simulink model "gmp_pmsm_sensored_nonlinear_sil_mdl_2022b"  (R2022b)
settings: Solver=VariableStepAuto  StartTime=0.0  StopTime=10  RelTol=1e-3
model workspace (MAT data in the model file):
  B = 0
  BW_i = 800
  Flux_t = 0.12
  IQ24 : Simulink.NumericType (value not decoded)
  J = 0.018
  K_d = 3.72061852168
  K_m = 0.128242020589
  K_u = 0.00236407598332
  Ki_id = 0.001
  Ki_iq = 1
  Ki_n = 25225.1136556
  Kp_id = 1e-05
  Kp_iq = 5e-05
  Kp_n = 12.6125568278
  Ld_t = 0.00303
  Lq_t = 0.02019
  Max_p = 0.006000830667
  P = 2
  RLS_ini_a = 1000000
  Rd_mos = 0.01
  Rs = 0.1215
  Rv = 6.4
  T_final = 0
  T_initial = 0
  Tes = [4 7 10 7 4]
  Tf_t = 0.1
  Tm = 0
  Udq_limit = 550
  Var = 0
  Vce0 = 0
  Vd0 = 0
  Vdc = 80
  button = 1
  im_limit = 40
  mean_prd = 10
  position_init = 0.2
  r_ce = 1e-08
  r_d = 1e-08
  sample_prd = 100
  step_time = 0.2
  ts = 6.25e-05
  wc = 3500
libraries: peripheral_utilities x9, spsSeriesRLCBranchLib x6, spsMosfetLib x6, simulink x3, spsVoltageMeasurementLib x2, gmp_sil_core_pack x1, spsPermanentMagnetSynchronousMachineLib x1, spsdq0toabcLib x1, spsFourierLib x1, spsControlledVoltageSourceLib x1, sps_lib x1
(part 2 of 3)

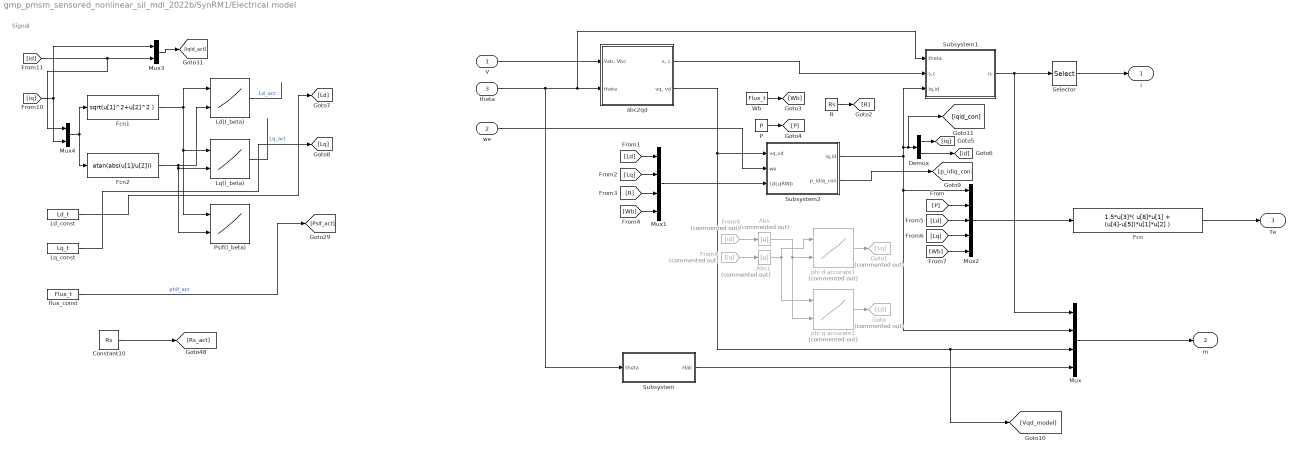
== system gmp_pmsm_sensored_nonlinear_sil_mdl_2022b/SynRM1/Electrical model ==
  note: Signal
  V : Inport
  we : Inport  Port=2
  theta : Inport  Port=3
  Abs : Abs  Commented=on  SaturateOnIntegerOverflow=off
  Abs1 : Abs  Commented=on  SaturateOnIntegerOverflow=off
  Constant10 : Constant  Value=Rs
  Demux : Demux  Outputs=2
  Fcn : Fcn  Expr=1.5*u[3]*( u[6]*u[1] + (u[4]-u[5])*u[1]*u[2] )
  Fcn1 : Fcn  Expr=sqrt(u[1]^2+u[2]^2 )
  Fcn2 : Fcn  Expr=atan(abs(u[1]/u[2]))
  From8 : From  Commented=on  GotoTag=iq
  From9 : From  Commented=on  GotoTag=id
  Goto : Goto  Commented=on  GotoTag=Ld
  Goto1 : Goto  Commented=on  GotoTag=Lq
  Ld(I_beta) : Lookup_n-D  BreakpointsForDimension1=[0,4,8,12,16,20,24,28,32,36,40,44,48,52,56,60,64,68,72,76]  BreakpointsForDimension2=[0,4,8,12,16,20,24,28,32,36,40,44,48,52,56,60,64,68,72,76,80,84,88,90]  Table=[0.0090049,0.0090049,0.0090049,0.0090049,0.0090049,0.0090049,0.0090049,0.0090049,0.0090049,0.0090049,0.0090049,0.0090049,0.0090049,0.0090049,0.0090049,0.0090049,0.0090049,0.0090049,0.0090049,0.0090049,0.0090049,0.0090049,0.0090049,0.0090049;0.0091068,0.0083359,0.0077182,0.0071952,0.0067602,0.0063986,0.0061075,0.0058615,0.0056442,0.0054621,0.0053073,0.0051722,0.0050586,0.0049576,0.0048709,0.0047948,0.0047272,0.0046738,0.0046308,0.0045967,0.00457,0.0045527,0.0045425,0.0045403;0.0093464,0.0079938,0.0070425,0.006355,0.0058504,0.0054685,0.005168,0.004922,0.0047173,0.0045442,0.0044053,0.0042808,0.0041752,0.0040816,0.0040014,0.0039315,0.0038713,0.0038189,0.0037747,0.0037414,0.0037159,0.0036999,0.0036913,0.0036904;0.0094184,0.0086648,0.007532,0.0065799,0.0059032,0.0053778,0.0049522,0.0046235,0.0043749,0.0041848,0.0040338,0.0039102,0.0038062,0.0037163,0.0036343,0.0035659,0.003505,0.0034522,0.0034077,0.003372,0.0033446,0.0033271,0.0033182,0.003317;0.007537,0.0073523,0.0068251,0.0060935,0.0054955,0.0050421,0.0046797,0.0043924,0.0041627,0.0039813,0.0038382,0.003715,0.0036051,0.0035122,0.0034334,0.0033641,0.0033014,0.0032455,0.0031985,0.00316,0.0031309,0.0031118,0.0031022,0.0031011;0.0069136,0.0066119,0.0061429,0.0055601,0.0050595,0.0046689,0.004363,0.0041106,0.0039094,0.0037548,0.0036311,0.0035297,0.003445,0.0033686,0.0032942,0.0032267,0.0031671,0.0031114,0.0030613,0.0030204,0.0029894,0.002969,0.0029587,0.0029574;0.0067888,0.0062678,0.005688,0.0051372,0.0047121,0.0043706,0.0040971,0.0038745,0.0037001,0.0035638,0.0034559,0.0033682,0.0032948,0.0032327,0.0031761,0.0031194,0.0030631,0.0030118,0.0029628,0.0029201,0.0028873,0.0028657,0.002855,0.0028536;0.0064852,0.0059179,0.0053416,0.0048215,0.0044208,0.0041168,0.0038718,0.0036757,0.0035267,0.0034084,0.0033126,0.0032335,0.0031693,0.0031162,0.0030692,0.0030242,0.0029766,0.0029286,0.0028841,0.0028423,0.0028087,0.0027864,0.0027753,0.0027739;0.0061523,0.0056113,0.0050565,0.0045719,0.0041984,0.0039199,0.0036926,0.0035158,0.0033808,0.0032752,0.0031919,0.0031227,0.0030647,0.0030165,0.0029765,0.0029393,0.0029008,0.0028583,0.002817,0.002778,0.0027453,0.0027227,0.0027115,0.0027103;0.0058954,0.0053596,0.0048097,0.0043561,0.0040148,0.0037503,0.0035417,0.0033833,0.0032591,0.0031631,0.0030877,0.0030266,0.0029757,0.0029326,0.0028962,0.0028645,0.0028327,0.0027967,0.0027584,0.0027223,0.002691,0.0026694,0.0026587,0.0026572;0.0056976,0.0051489,0.0045961,0.004167,0.0038525,0.0036066,0.0034122,0.0032677,0.0031545,0.0030661,0.0029972,0.0029426,0.0028976,0.0028598,0.0028271,0.0027991,0.0027724,0.0027421,0.002707,0.0026731,0.0026436,0.0026234,0.0026135,0.0026121;0.0055231,0.0049627,0.0044187,0.0040007,0.0037069,0.0034785,0.0032983,0.0031643,0.0030617,0.0029804,0.0029182,0.0028686,0.0028288,0.0027956,0.0027666,0.0027417,0.0027187,0.0026929,0.0026618,0.0026296,0.0026011,0.0025825,0.0025738,0.0025727;0.0053694,0.0047911,0.0042535,0.0038565,0.0035785,0.0033645,0.0031988,0.0030752,0.0029797,0.0029055,0.0028481,0.0028031,0.002767,0.0027377,0.002713,0.0026907,0.0026708,0.0026487,0.0026213,0.0025909,0.0025632,0.0025454,0.0025381,0.0025373;0.0052237,0.0046319,0.0041064,0.0037302,0.0034662,0.0032628,0.0031101,0.0029956,0.0029078,0.0028387,0.0027859,0.0027449,0.0027117,0.0026861,0.0026645,0.0026452,0.0026275,0.0026087,0.0025847,0.002556,0.0025292,0.0025117,0.0025053,0.0025047;0.0050914,0.0044851,0.003973,0.0036151,0.0033625,0.0031734,0.0030322,0.0029247,0.0028431,0.0027797,0.0027305,0.0026924,0.0026625,0.0026388,0.0026201,0.002604,0.0025886,0.0025725,0.0025511,0.0025243,0.0024983,0.0024809,0.0024746,0.0024742;0.004977,0.004351,0.0038492,0.0035074,0.0032708,0.0030953,0.0029629,0.0028607,0.0027852,0.0027265,0.002681,0.0026455,0.0026177,0.0025961,0.0025796,0.0025663,0.0025528,0.0025391,0.0025203,0.0024953,0.00247,0.0024526,0.002446,0.0024453;0.0048627,0.0042246,0.0037365,0.0034117,0.0031881,0.0030249,0.0028998,0.002804,0.0027327,0.0026783,0.0026359,0.0026029,0.0025771,0.0025573,0.0025427,0.0025312,0.0025199,0.0025084,0.0024918 ...(+761 chars)]  InterpMethod=Akima spline  RndMeth=Simplest
      settings: InputPortMap=u0,u1
  Ld_const : Constant  Value=Ld_t
  Lq(I_beta) : Lookup_n-D  BreakpointsForDimension1=[0,4,8,12,16,20,24,28,32,36,40,44,48,52,56,60,64,68,72,76]  BreakpointsForDimension2=[0,4,8,12,16,20,24,28,32,36,40,44,48,52,56,60,64,68,72,76,80,84,88,90]  Table=[0.027272,0.027272,0.027272,0.027272,0.027272,0.027272,0.027272,0.027272,0.027272,0.027272,0.027272,0.027272,0.027272,0.027272,0.027272,0.027272,0.027272,0.027272,0.027272,0.027272,0.027272,0.027272,0.027272,0.027272;0.027457,0.027451,0.027443,0.027434,0.027425,0.027414,0.027402,0.02739,0.027376,0.027361,0.027345,0.027328,0.027312,0.027294,0.027277,0.02726,0.027243,0.027228,0.027214,0.027202,0.027193,0.027187,0.027183,0.027183;0.027424,0.02742,0.027429,0.027443,0.027463,0.027488,0.027502,0.027506,0.027502,0.027489,0.02747,0.027448,0.02742,0.027389,0.027353,0.027315,0.027274,0.027232,0.02719,0.027153,0.027123,0.027102,0.027091,0.02709;0.024416,0.024514,0.024663,0.024863,0.025117,0.025413,0.025742,0.02607,0.026395,0.026688,0.026936,0.027154,0.027312,0.027386,0.02738,0.027348,0.027301,0.027245,0.027182,0.027117,0.027059,0.027015,0.026992,0.026989;0.02017,0.02027,0.02045,0.020689,0.02099,0.021369,0.02182,0.022355,0.022972,0.023672,0.024447,0.025225,0.025912,0.02649,0.026932,0.027211,0.027268,0.027228,0.027161,0.02708,0.026997,0.026928,0.026888,0.026883;0.017083,0.017167,0.017325,0.017546,0.017836,0.018192,0.018626,0.019145,0.019755,0.020476,0.021306,0.02226,0.023328,0.024442,0.025444,0.02627,0.026871,0.027127,0.027109,0.027029,0.026931,0.026839,0.026782,0.026775;0.014717,0.014798,0.014939,0.015143,0.015413,0.015756,0.016171,0.016667,0.017254,0.017938,0.018741,0.019678,0.02076,0.022,0.023359,0.024679,0.025792,0.026628,0.026978,0.026954,0.026855,0.026746,0.026674,0.026664;0.012887,0.012961,0.013093,0.013279,0.013524,0.013837,0.014221,0.014684,0.015243,0.015903,0.016678,0.017574,0.018624,0.019853,0.021269,0.022834,0.024363,0.025653,0.026571,0.02683,0.026764,0.026648,0.026562,0.026551;0.011447,0.011518,0.01164,0.011811,0.012035,0.012323,0.012674,0.013102,0.013617,0.014233,0.014972,0.015841,0.016854,0.018037,0.019437,0.021055,0.022814,0.024466,0.025829,0.026582,0.026648,0.026543,0.026448,0.026435;0.010299,0.010364,0.010475,0.010633,0.010841,0.011105,0.011431,0.011827,0.012302,0.012874,0.013559,0.01438,0.015359,0.016508,0.01786,0.019466,0.021308,0.023214,0.02491,0.026137,0.026485,0.026425,0.026329,0.026314;0.009364,0.0094217,0.0095231,0.0096707,0.0098639,0.010107,0.010408,0.010777,0.01122,0.011752,0.012391,0.013158,0.014081,0.015193,0.016508,0.018073,0.019924,0.021976,0.023923,0.025531,0.026262,0.02629,0.026204,0.026188;0.0085868,0.0086393,0.0087346,0.0088688,0.0090479,0.0092749,0.0095542,0.0098959,0.010311,0.010809,0.011409,0.01213,0.013,0.014056,0.015331,0.016852,0.018681,0.020793,0.022941,0.024838,0.025951,0.026132,0.02607,0.026056;0.0079329,0.0079796,0.0080672,0.0081916,0.0083583,0.0085706,0.008832,0.0091518,0.0095399,0.010008,0.010572,0.011251,0.012073,0.013074,0.014298,0.015777,0.017569,0.019694,0.021981,0.024103,0.025573,0.025947,0.025924,0.025914;0.0073732,0.0074161,0.0074969,0.0076131,0.0077693,0.0079668,0.0082118,0.0085126,0.0088775,0.0093177,0.0098501,0.010494,0.011271,0.012223,0.013393,0.014827,0.016573,0.018688,0.021065,0.023353,0.02514,0.025741,0.025766,0.02576;0.0068903,0.0069293,0.0070039,0.0071128,0.0072591,0.0074446,0.0076753,0.0079587,0.008303,0.0087195,0.0092225,0.0098328,0.010572,0.011476,0.012594,0.013981,0.015681,0.017769,0.020191,0.022618,0.024668,0.025516,0.025595,0.025593;0.0064698,0.0065049,0.006574,0.006676,0.0068138,0.006989,0.0072071,0.0074741,0.0078002,0.0081951,0.008673,0.0092517,0.009955,0.010818,0.011886,0.013225,0.014879,0.016928,0.019366,0.021908,0.024161,0.025263,0.025412,0.025411;0.0060997,0.0061318,0.0061962,0.006292,0.0064219,0.0065878,0.006794,0.0070472,0.0073565,0.0077323,0.0081866,0.0087375,0.0094085,0.010233,0.011257,0.012545,0.014154,0.01616,0.018596,0.021224,0.023646,0.024992,0.025219,0.025221;0.0057719,0.0058012,0.0058613,0.0059518,0.0060743,0.006232,0.0064275,0.0066679,0.0069624,0.0073201,0.0077535,0.0082795,0.0089208,0.0097104,0.010693,0.011932,0.013497,0.015458,0.017879,0.020565,0.023132,0.024704,0.025018,0.025025;0.0054794,0.0055061,0.0055623,0.0056477,0.0057645,0.0059136,0.0060997,0.0063293,0.0066096,0.0069515,0.0073655,0.0078687,0.0084832,0.0092404,0.010185,0.011379,0.012899,0.014818,0.017211,0.01994,0.022622,0.024403,0.02481,0.024823;0.0052168,0.0052407,0.005294,0.0053748,0.0054858,0.0056282,0.0058054,0.0060247,0.0062924,0.0066197,0.0070165,0.0074986,0.0080883,0.0088162,0.0097256,0.010878,0.012353,0.014228,0.016589,0.019344,0.022118,0.024093,0.024597,0.024612]  InterpMethod=Akima spline  RndMeth=Simplest
      settings: InputPortMap=u0,u1
  Lq_const : Constant  Value=Lq_t
  Mux : Mux  Inputs=[3, 2, 2, 3]
  Mux1 : Mux
  Mux2 : Mux  Inputs=[2, 1, 1, 1, 1]
  Mux3 : Mux  Inputs=2
  Mux4 : Mux  Inputs=2
  P : Constant  Value=P
  Psif(I_beta) : Lookup_n-D  BreakpointsForDimension1=[0,4,8,12,16,20,24,28,32,36,40,44,48,52,56,60,64,68,72,76]  BreakpointsForDimension2=[0,4,8,12,16,20,24,28,32,36,40,44,48,52,56,60,64,68,72,76,80,84,88,90]  Table=[0.098812,0.098812,0.098812,0.098812,0.098812,0.098812,0.098812,0.098812,0.098812,0.098812,0.098812,0.098812,0.098812,0.098812,0.098812,0.098812,0.098812,0.098812,0.098812,0.098812,0.098812,0.098812,0.098812,0.098812;0.10048,0.10244,0.104,0.10523,0.10621,0.107,0.10765,0.10817,0.10856,0.10888,0.10913,0.10932,0.10947,0.10958,0.10965,0.10969,0.10969,0.10971,0.10973,0.10973,0.10973,0.10972,0.10971,0.1097;0.10442,0.10813,0.11059,0.11225,0.1134,0.11418,0.11469,0.11497,0.11508,0.11505,0.11497,0.11478,0.11455,0.11425,0.11394,0.11362,0.1133,0.11298,0.11269,0.11247,0.11229,0.11217,0.1121,0.1121;0.10971,0.11589,0.11975,0.12184,0.12303,0.12353,0.12346,0.12308,0.12254,0.12191,0.12121,0.12046,0.11969,0.11884,0.11791,0.11705,0.11621,0.11543,0.11474,0.11417,0.11372,0.11342,0.11326,0.11324;0.11029,0.11747,0.12299,0.12605,0.12777,0.12873,0.12907,0.12908,0.12884,0.12842,0.12784,0.12689,0.12548,0.1239,0.12233,0.12077,0.11924,0.11782,0.11659,0.11556,0.11476,0.11423,0.11396,0.11393;0.11005,0.11803,0.12418,0.1279,0.13009,0.13139,0.13209,0.1323,0.13224,0.13209,0.13177,0.13124,0.13044,0.12915,0.12715,0.12485,0.12259,0.12041,0.11846,0.11687,0.11566,0.11485,0.11445,0.11439;0.10978,0.11858,0.12492,0.12891,0.13157,0.13321,0.13416,0.13462,0.13482,0.13483,0.13469,0.13436,0.13378,0.13288,0.13145,0.12917,0.12624,0.12328,0.12051,0.11822,0.1165,0.11537,0.11481,0.11474;0.10932,0.11886,0.12552,0.12974,0.13252,0.1344,0.13556,0.13626,0.13681,0.13714,0.13722,0.137,0.13656,0.13585,0.13471,0.13287,0.12998,0.12637,0.1228,0.11966,0.11734,0.11583,0.1151,0.115;0.10852,0.11876,0.12585,0.13038,0.13338,0.1355,0.1368,0.1377,0.13841,0.13893,0.1393,0.13937,0.13908,0.13845,0.13747,0.13588,0.13333,0.12955,0.12529,0.12125,0.11819,0.11624,0.1153,0.11519;0.10747,0.11845,0.12586,0.13067,0.13398,0.13623,0.13777,0.13896,0.13984,0.14054,0.14107,0.14137,0.14135,0.14089,0.13996,0.13851,0.1362,0.13254,0.12779,0.12296,0.119,0.11653,0.11537,0.11522;0.10635,0.118,0.12564,0.13073,0.13433,0.13678,0.1385,0.13993,0.14105,0.14195,0.14265,0.14314,0.14333,0.14311,0.14231,0.14092,0.13874,0.13521,0.13016,0.12474,0.11993,0.11686,0.11543,0.11524;0.10517,0.11745,0.12541,0.13063,0.13445,0.13713,0.13904,0.14067,0.14207,0.14317,0.1441,0.14476,0.14513,0.14511,0.14451,0.14318,0.14104,0.13763,0.13254,0.12656,0.12096,0.11718,0.11545,0.11523;0.10395,0.11682,0.12504,0.13049,0.13447,0.13734,0.13953,0.14139,0.14297,0.14431,0.14543,0.14626,0.14676,0.14689,0.14651,0.14529,0.14325,0.13995,0.13486,0.12838,0.12203,0.11753,0.11544,0.11519;0.10276,0.11613,0.12463,0.13031,0.13449,0.1375,0.13993,0.14203,0.14384,0.14536,0.14667,0.14768,0.1483,0.14859,0.14836,0.14735,0.14535,0.14212,0.13702,0.13016,0.12313,0.11787,0.11539,0.11509;0.10156,0.1154,0.12417,0.13005,0.13438,0.13766,0.14035,0.14264,0.14468,0.14641,0.14787,0.14904,0.14982,0.1502,0.15009,0.14928,0.14738,0.14419,0.13906,0.1319,0.12425,0.11823,0.11534,0.11499;0.10039,0.11469,0.12364,0.12971,0.13429,0.13787,0.14078,0.14323,0.14549,0.14744,0.14908,0.15039,0.15131,0.15178,0.15177,0.15112,0.14932,0.14616,0.14103,0.13362,0.12538,0.11863,0.11529,0.11488;0.099234,0.11395,0.1231,0.12941,0.13422,0.13808,0.14119,0.14387,0.1463,0.14848,0.15028,0.15174,0.15277,0.15335,0.15345,0.15289,0.15121,0.1481,0.14294,0.13532,0.12653,0.11904,0.11523,0.11476;0.098088,0.11321,0.12261,0.12916,0.1342,0.13832,0.14162,0.14454,0.14714,0.1495,0.15149,0.15309,0.15423,0.15493,0.15508,0.15462,0.15305,0.14998,0.14482,0.137,0.1277,0.11947,0.11519,0.11465;0.096962,0.11249,0.12213,0.12891,0.13424,0.13858,0.1421,0.14524,0.14802,0.15058,0.15273,0.15446,0.15571,0.15649,0.15674,0.15633,0.15488,0.15185,0.14667,0.13866,0.12887,0.11989,0.11508,0.11448;0.095857,0.11178,0.12171,0.12869,0.13431,0.13891,0.14261,0.14597,0.14896,0.1517,0.15401,0.15587,0.15722,0.15808,0.15838,0.15803,0.1567,0.15371,0.14849,0.14029,0.12999,0.12027,0.11494,0.11428]  InterpMethod=Akima spline  RndMeth=Simplest
      settings: InputPortMap=u0,u1
  R : Constant  Value=Rs
  Selector : Selector  InputPortWidth=3  IndexOptions=Index vector (dialog)  Indices=[1 2]  OutputSizes=1
  Subsystem : Subsystem
  Subsystem1 : Subsystem
  Subsystem2 : Subsystem
  Wb : Constant  Value=Flux_t
  abc2qd : Subsystem
  flux_const : Constant  Value=Flux_t
  phi d accurate1 : Lookup_n-D  Commented=on  BreakpointsForDimension1="[0     3     6     9    12    15    18    21    24    27    30]"  BreakpointsForDimension2="[0     3     6     9    12    15    18    21    24    27    30]"  Table=|  RndMeth=Simplest
      | [0.0227	0.0222	0.021833333	0.0215	0.021233333	0.021	0.0208	0.020633333	0.0205	0.020366667	0.0202;
      | 0.0227	0.0222	0.021833333	0.0215	0.021233333	0.021	0.0208	0.020633333	0.0205	0.020366667	0.0202;
      | 0.02265	0.022283333	0.021916667	0.0216	0.021333333	0.021083333	0.020883333	0.020683333	0.0205	0.020283333	0.02005;
      | 0.022433333	0.022144444	0.021822222	0.021522222	0.021244444	0.020977778	0.020711111	0.020433333	0.020144444	0.019844444	0.019511111;
      | 0.021375	0.021183333	0.020916667	0.020641667	0.020358333	0.020066667	0.019758333	0.019425	0.019075	0.018708333	0.018316667;
      | 0.0192	0.019106667	0.01894	0.01874	0.01852	0.018273333	0.018006667	0.01772	0.017413333	0.017086667	0.01674;
      | 0.0171	0.017055556	0.01695	0.016811111	0.01665	0.016461111	0.016255556	0.016033333	0.015788889	0.015522222	0.015244444;
      | 0.01537619	0.015347619	0.015280952	0.015180952	0.015061905	0.014919048	0.014757143	0.014580952	0.014385714	0.01417619	0.013957143;
      | 0.013979167	0.0139625	0.0139125	0.013841667	0.013745833	0.0136375	0.013508333	0.013366667	0.0132125	0.013041667	0.0128625;
      | 0.012833333	0.012818519	0.012785185	0.01272963	0.012659259	0.01257037	0.012466667	0.012351852	0.012225926	0.012085185	0.011937037;
      | 0.011876667	0.011866667	0.01184	0.011796667	0.01174	0.01167	0.011586667	0.01149	0.011386667	0.01127	0.011146667;]
      settings: InputPortMap=u0,u1
  phi q accurate1 : Lookup_n-D  Commented=on  BreakpointsForDimension1="[0     3     6     9    12    15    18    21    24    27    30]"  BreakpointsForDimension2="[0     3     6     9    12    15    18    21    24    27    30]"  Table=|  RndMeth=Simplest
      | [0.010733333	0.010733333	0.00825	0.007344444	0.006841667	0.00652	0.0063	0.006133333	0.006004167	0.0059	0.005816667;
      | 0.0105	0.0105	0.008183333	0.007288889	0.006808333	0.0065	0.006283333	0.00612381	0.005995833	0.005896296	0.005806667;
      | 0.009833333	0.009833333	0.007916667	0.007144444	0.006716667	0.006433333	0.006238889	0.006085714	0.005966667	0.005866667	0.005776667;
      | 0.008966667	0.008966667	0.007516667	0.0069	0.00655	0.006313333	0.006138889	0.006	0.0058875	0.005788889	0.0057;
      | 0.0079	0.0079	0.007016667	0.006566667	0.0063	0.006113333	0.005966667	0.005842857	0.005741667	0.005648148	0.005563333;
      | 0.007033333	0.007033333	0.0065	0.0062	0.006	0.005853333	0.005738889	0.005638095	0.00555	0.005466667	0.005393333;
      | 0.006433333	0.006433333	0.006083333	0.005877778	0.005725	0.005606667	0.005511111	0.005428571	0.005354167	0.005285185	0.005216667;
      | 0.006033333	0.006033333	0.00575	0.005588889	0.005475	0.005386667	0.005305556	0.005233333	0.005170833	0.005111111	0.00505;
      | 0.0057	0.0057	0.005483333	0.005355556	0.005258333	0.005186667	0.005116667	0.005057143	0.005	0.004948148	0.004896667;
      | 0.005433333	0.005433333	0.005266667	0.005144444	0.005066667	0.005	0.004944444	0.004895238	0.004845833	0.0048	0.004753333;
      | 0.005233333	0.005233333	0.005083333	0.004966667	0.004891667	0.00484	0.004788889	0.004747619	0.004704167	0.004659259	0.00462;]
      settings: InputPortMap=u0,u1
  i : Outport  VectorParamsAs1DForOutWhenUnconnected=off
  m : Outport  Port=2  VectorParamsAs1DForOutWhenUnconnected=off
  Te : Outport  Port=3  VectorParamsAs1DForOutWhenUnconnected=off
  wires:
  V/1 -> abc2qd/1("Vab, Vbc")
  theta/1 -> Subsystem/1(theta), Subsystem1/1(theta), abc2qd/2(theta)
  Subsystem2/1(iq,id) -> Mux2/1, Mux/2, [iqid_con], Demux/1, Subsystem1/3(iq,id)
  Wb/1 -> [Wb]
  we/1 -> Subsystem2/2(we)
  abc2qd/1("s, c") -> Subsystem1/2(s,c)
  [Lq] -> Mux1/2
  P/1 -> [P]
  Mux1/1 -> Subsystem2/3(LdLqRWb)
  [Wb] -> Mux2/5
  Mux2/1 -> Fcn/1
  R/1 -> [R]
  [Ld] -> Mux1/1
  Fcn/1 -> Te/1
  abc2qd/2("vq, vd") -> [Vqd_model], Mux/3, Subsystem2/1(vq,vd)
  [Ld] -> Mux2/3
  Mux/1 -> m/1
  Subsystem1/1(is) -> Mux/1, Selector/1
  Selector/1 -> i/1
  [R] -> Mux1/3
  Subsystem/1(Hall) -> Mux/4
  [P] -> Mux2/2
  [Lq] -> Mux2/4
  [Wb] -> Mux1/4
  Demux/2 -> [id]
  Demux/1 -> [iq]
  Abs/1 -> phi q accurate1/2, phi d accurate1/2
  phi q accurate1/1 -> Goto/1
  Abs1/1 -> phi q accurate1/1, phi d accurate1/1
  phi d accurate1/1 -> Goto1/1
  From8/1 -> Abs1/1
  From9/1 -> Abs/1
  Ld(I_beta)/1 -> ?  "Ld_act"
  Mux3/1 -> [iqid_act]
  Constant10/1 -> [Rs_act]
  [iq] -> Mux3/1, Mux4/2
  Lq(I_beta)/1 -> ?  "Lq_act"
  flux_const/1 -> [Psif_act]  "phif_act"
  [id] -> Mux3/2, Mux4/1
  Subsystem2/2(p_idiq_con) -> [p_idiq_con]
  Mux4/1 -> Fcn2/1, Fcn1/1
  Fcn1/1 -> Ld(I_beta)/1, Psif(I_beta)/1, Lq(I_beta)/1
  Fcn2/1 -> Psif(I_beta)/2, Lq(I_beta)/2, Ld(I_beta)/2
  Ld_const/1 -> [Ld]
  Lq_const/1 -> [Lq]

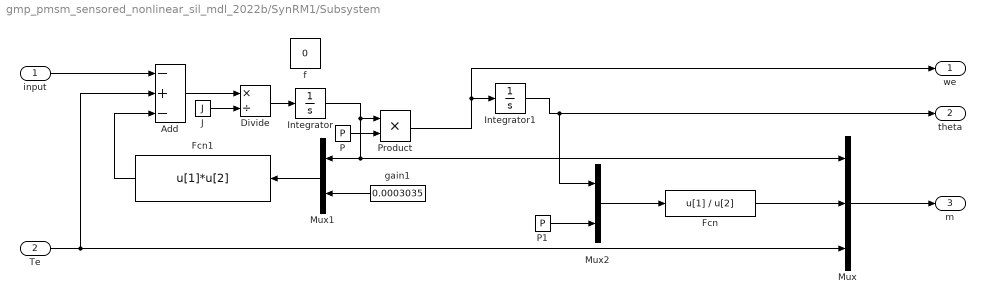
== system gmp_pmsm_sensored_nonlinear_sil_mdl_2022b/SynRM1/Subsystem ==
  input : Inport
  Te : Inport  Port=2
  Add : Sum  Inputs=-+-
  Divide : Product  Inputs=*/
  Fcn : Fcn  Expr=u[1] / u[2]
  Fcn1 : Fcn  Expr=u[1]*u[2]
  Integrator : Integrator
  Integrator1 : Integrator  InitialCondition=position_init
  J : Constant  Value=J  VectorParams1D=off
  Mux : Mux  Inputs=3
  Mux1 : Mux  Inputs=2
  Mux2 : Mux  Inputs=2
  P : Constant  Value=P
  P1 : Constant  Value=P
  Product : Product
  f : Constant  Value=0
  gain1 : Constant  Value=0.0003035
  we : Outport  VectorParamsAs1DForOutWhenUnconnected=off
  theta : Outport  Port=2  VectorParamsAs1DForOutWhenUnconnected=off
  m : Outport  Port=3  VectorParamsAs1DForOutWhenUnconnected=off
  wires:
  input/1 -> Add/1
  Te/1 -> Mux/3, Add/2
  J/1 -> Divide/2
  Add/1 -> Divide/1
  Divide/1 -> Integrator/1
  P/1 -> Product/2
  Integrator/1 -> Mux/1, Mux1/1, Product/1
  Integrator1/1 -> Mux2/1, theta/1
  Mux/1 -> m/1
  Mux1/1 -> Fcn1/1
  Fcn1/1 -> Add/3
  Mux2/1 -> Fcn/1
  Fcn/1 -> Mux/2
  P1/1 -> Mux2/2
  gain1/1 -> Mux1/2
  Product/1 -> we/1, Integrator1/1

== system gmp_pmsm_sensored_nonlinear_sil_mdl_2022b/SynRM1/Subsystem1 ==
  m_e : Inport
  m_m : Inport  Port=2
  Bus Creator : BusCreator  Inputs=13
  Demux : Demux  Outputs=[1, 1, 1]
  Demux1 : Demux  Outputs=[1, 1, 1, 1, 1, 1, 1, 1, 1, 1]
  Out : Outport  VectorParamsAs1DForOutWhenUnconnected=off
  wires:
  Demux1/1 -> Bus Creator/1  "Stator current is_a (A)"
  Demux1/2 -> Bus Creator/2  "Stator current is_b (A)"
  Demux1/3 -> Bus Creator/3  "Stator current is_c (A)"
  Demux1/4 -> Bus Creator/4  "Stator current is_q (A)"
  Demux1/5 -> Bus Creator/5  "Stator current is_d (A)"
  Demux1/6 -> Bus Creator/6  "Stator voltage Vs_q (V)"
  Demux1/7 -> Bus Creator/7  "Stator voltage Vs_d (V)"
  Demux1/8 -> Bus Creator/8  "Hall effect signal h_a"
  Demux1/9 -> Bus Creator/9  "Hall effect signal h_b"
  Demux1/10 -> Bus Creator/10  "Hall effect signal h_c"
  Demux/1 -> Bus Creator/11  "Rotor speed wm (rad/s)"
  Demux/2 -> Bus Creator/12  "Rotor angle thetam (rad)"
  Demux/3 -> Bus Creator/13  "Electromagnetic torque Te (N*m)"
  Bus Creator/1 -> Out/1
  m_m/1 -> Demux/1
  m_e/1 -> Demux1/1

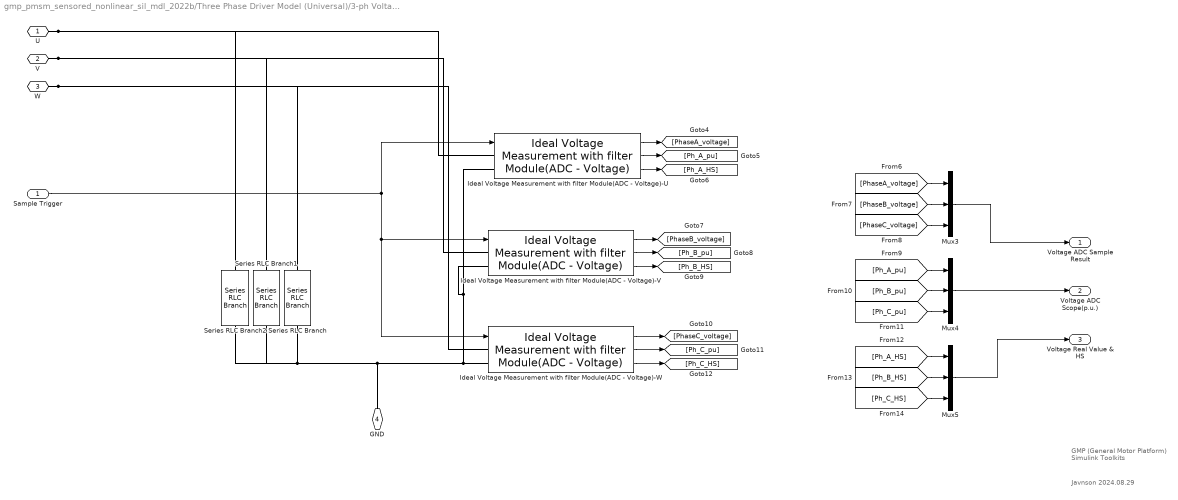
== system gmp_pmsm_sensored_nonlinear_sil_mdl_2022b/Three Phase Driver Model (Universal)/3-ph Voltage measurement ==
  note: Javnson
      | 2024.08.29
  note: GMP (General Motor Platform)
      | Simulink Toolkits
  Sample Trigger : Inport
  Ideal Voltage Measurement with filter Module(ADC - Voltage)-U : peripheral_utilities/Ideal Voltage Measurement with filter Module(ADC - Voltage)  ADC_GAIN=ADC_GAIN  ADC_BIT=ADC_BIT  ADC_REFERENCE=ADC_REFERENCE  ADC_BIAS=ADC_BIAS  ADC_INIT=ADC_INIT  cut_frequency=cut_frequency
      settings: SourceProductName=GMP Utilities Library
  Ideal Voltage Measurement with filter Module(ADC - Voltage)-V : peripheral_utilities/Ideal Voltage Measurement with filter Module(ADC - Voltage)  ADC_GAIN=ADC_GAIN  ADC_BIT=ADC_BIT  ADC_REFERENCE=ADC_REFERENCE  ADC_BIAS=ADC_BIAS  ADC_INIT=ADC_INIT  cut_frequency=cut_frequency
      settings: SourceProductName=GMP Utilities Library
  Ideal Voltage Measurement with filter Module(ADC - Voltage)-W : peripheral_utilities/Ideal Voltage Measurement with filter Module(ADC - Voltage)  ADC_GAIN=ADC_GAIN  ADC_BIT=ADC_BIT  ADC_REFERENCE=ADC_REFERENCE  ADC_BIAS=ADC_BIAS  ADC_INIT=ADC_INIT  cut_frequency=cut_frequency
      settings: SourceProductName=GMP Utilities Library
  Mux3 : Mux  Inputs=3
  Mux4 : Mux  Inputs=3
  Mux5 : Mux  Inputs=3
  Series RLC Branch : spsSeriesRLCBranchLib/Series RLC Branch  LConnTagsString=__new0  RConnTagsString=__new0  BranchType=R  Resistance=1e6  Inductance=1e-3  SetiL0=off  InitialCurrent=0  Capacitance=1e-6  Setx0=off  InitialVoltage=0  Measurements=None
  Series RLC Branch1 : spsSeriesRLCBranchLib/Series RLC Branch  LConnTagsString=__new0  RConnTagsString=__new0  BranchType=R  Resistance=1e6  Inductance=1e-3  SetiL0=off  InitialCurrent=0  Capacitance=1e-6  Setx0=off  InitialVoltage=0  Measurements=None
  Series RLC Branch2 : spsSeriesRLCBranchLib/Series RLC Branch  LConnTagsString=__new0  RConnTagsString=__new0  BranchType=R  Resistance=1e6  Inductance=1e-3  SetiL0=off  InitialCurrent=0  Capacitance=1e-6  Setx0=off  InitialVoltage=0  Measurements=None
  U : PMIOPort  Side=Left
  V : PMIOPort  Port=2  Side=Left
  W : PMIOPort  Port=3  Side=Left
  GND : PMIOPort  Port=4  Side=Left
  Voltage ADC Sample Result : Outport
  Voltage ADC Scope(p.u.) : Outport  Port=2
  Voltage Real Value & HS : Outport  Port=3
  wires:
  Ideal Voltage Measurement with filter Module(ADC - Voltage)-W/3 -> [Ph_C_HS]
  Sample Trigger/1 -> Ideal Voltage Measurement with filter Module(ADC - Voltage)-U/1, Ideal Voltage Measurement with filter Module(ADC - Voltage)-W/1, Ideal Voltage Measurement with filter Module(ADC - Voltage)-V/1
  Ideal Voltage Measurement with filter Module(ADC - Voltage)-V/2 -> [Ph_B_pu]
  Ideal Voltage Measurement with filter Module(ADC - Voltage)-V/3 -> [Ph_B_HS]
  Mux4/1 -> Voltage ADC Scope(p.u.)/1
  [Ph_B_HS] -> Mux5/2
  Ideal Voltage Measurement with filter Module(ADC - Voltage)-W/1 -> [PhaseC_voltage]
  Ideal Voltage Measurement with filter Module(ADC - Voltage)-V/1 -> [PhaseB_voltage]
  Ideal Voltage Measurement with filter Module(ADC - Voltage)-U/1 -> [PhaseA_voltage]
  Ideal Voltage Measurement with filter Module(ADC - Voltage)-U/2 -> [Ph_A_pu]
  [Ph_B_pu] -> Mux4/2
  [PhaseB_voltage] -> Mux3/2
  Ideal Voltage Measurement with filter Module(ADC - Voltage)-U/3 -> [Ph_A_HS]
  Ideal Voltage Measurement with filter Module(ADC - Voltage)-W/2 -> [Ph_C_pu]
  [Ph_A_pu] -> Mux4/1
  [PhaseC_voltage] -> Mux3/3
  [PhaseA_voltage] -> Mux3/1
  [Ph_C_pu] -> Mux4/3
  [Ph_C_HS] -> Mux5/3
  Mux3/1 -> Voltage ADC Sample Result/1
  [Ph_A_HS] -> Mux5/1
  Mux5/1 -> Voltage Real Value & HS/1
  connections:
  Ideal Voltage Measurement with filter Module(ADC - Voltage)-V/LConn2 -- Ideal Voltage Measurement with filter Module(ADC - Voltage)-U/LConn2 -- Series RLC Branch2/RConn1 -- Series RLC Branch1/RConn1 -- Series RLC Branch/RConn1 -- GND/RConn1 -- Ideal Voltage Measurement with filter Module(ADC - Voltage)-W/LConn2
  U/RConn1 -- Series RLC Branch2/LConn1 -- Ideal Voltage Measurement with filter Module(ADC - Voltage)-U/LConn1
  V/RConn1 -- Series RLC Branch1/LConn1 -- Ideal Voltage Measurement with filter Module(ADC - Voltage)-V/LConn1
  W/RConn1 -- Series RLC Branch/LConn1 -- Ideal Voltage Measurement with filter Module(ADC - Voltage)-W/LConn1

== system gmp_pmsm_sensored_nonlinear_sil_mdl_2022b/Three Phase Driver Model (Universal)/Single Phase Full Bridge U ==
  Enable : Inport
  PWM CMP : Inport  Port=2
  MOSFET LOWER : spsMosfetLib/Mosfet  Ron=R_mosfet_on  Lon=Lon  Rd=Rd  Vfd=Vf  IC=0  Rs=Rs  Cs=Cs  Measurements=off
  MOSFET UPPER : spsMosfetLib/Mosfet  Ron=R_mosfet_on  Lon=Lon  Rd=Rd  Vfd=Vf  IC=0  Rs=Rs  Cs=Cs  Measurements=off
  Triangle PWM modulation (with deadband)1 : Subsystem  mask{fswitch=fswitch, CMP_MAX=CMP_MAX, Deadband_Upper=Deadband_Upper, Deadband_Lower=Deadband_Lower, Deadband_us=NaN, phase_shift=phase_shift}
      mask prompts: Deadband_us "Deadband Time: (μs)"
      mask init:
      | calculate_deadband(gcb, 'Deadband_Upper', 'Deadband_Lower',	'CMP_MAX', 'fswitch', 'Deadband_us');
      mask Callback fswitch: calculate_deadband(gcb, 'Deadband_Upper', 'Deadband_Lower',	'CMP_MAX', 'fswitch', 'Deadband_us');
      mask Callback CMP_MAX: calculate_deadband(gcb, 'Deadband_Upper', 'Deadband_Lower',	'CMP_MAX', 'fswitch', 'Deadband_us');
      mask Callback Deadband_Upper:
      | calculate_deadband(gcb, 'Deadband_Upper', 'Deadband_Lower',	'CMP_MAX', 'fswitch', 'Deadband_us');
      | 
      | % Get handle of Mask
      | %mask_obj = Simulink.Mask.get(gcb);
      | %Parameters = Simulink.Mask.get(gcb).Parameters;
      | 
      | % Get source data
      | %dead_band_up = str2double(Parameters(strcmp(get_param(gcb,'MaskNames'),'Deadband_Upper')==1).Value);
      | %dead_band_dn = str2double(Parameters(strcmp(get_param(gcb,'MaskNames'),'Deadband_Lower')==1).Value);
      | %cmp_max = str2double(Parameters(strcmp(get_param(gcb,'MaskNames'),'CMP_MAX')==1).Value);
      | %switch_freq = str2double(Parameters(strcmp(get_param(gcb,'MaskNames'),'fswitch')==1).Value);
      | 
      | % calculate deadband
      | %dead_band_us = 1/switch_freq * (dead_band_up + dead_band_dn) / cmp_max*1e6;
      | 
      | % Set result
      | %Parameters(strcmp(get_param(gcb,'MaskNames'),'Deadband_upper_us')==1).Value=num2str(dead_band_us);
      mask Callback Deadband_Lower: calculate_deadband(gcb, 'Deadband_Upper', 'Deadband_Lower',	'CMP_MAX', 'fswitch', 'Deadband_upper_us');
      mask DialogControl DescGroupVar Prompt: PWM Modulator
      mask DialogControl Control8 Prompt: GMP CTL Simulink Utilities: virtual peripherals
      mask DialogControl DescTextVar Prompt: PWM Modulator. Input PWM compare register value, output ADC trigger signal, PWM output and negtive PWM output.
      mask DialogControl ParameterGroupVar Prompt: 参数
      mask DialogControl Control2 Prompt: PWM Frequency (Hz) :
      mask DialogControl Control4 Prompt: Full Scale PWM Compare value:
      mask DialogControl Control5 Prompt: (whole period is 2 * CMP_MAX ticks)
      mask DialogControl Control3 Prompt: Deadband Range Set (CMP Value):
      mask DialogControl Control6 Prompt: Single side deadband time: DEADBAND_CMP/2/CMP_MAX/fswitch
      mask DialogControl Control7 Prompt: Initial Phase (rad)
  D : PMIOPort  Side=Left
  Phase : PMIOPort  Port=2  Side=Right
  S : PMIOPort  Port=3  Side=Right
  Sample Trigger Output : Outport
  wires:
  PWM CMP/1 -> Triangle PWM modulation (with deadband)1/2(PWM CMP)
  Triangle PWM modulation (with deadband)1/2(PWM OUTPUT N) -> MOSFET LOWER/1
  Triangle PWM modulation (with deadband)1/3(Sample Trigger Output) -> Sample Trigger Output/1
  Enable/1 -> Triangle PWM modulation (with deadband)1/1(Enable)
  Triangle PWM modulation (with deadband)1/1(PWM OUTPUT) -> MOSFET UPPER/1
  connections:
  MOSFET LOWER/RConn1 -- S/RConn1
  MOSFET UPPER/RConn1 -- Phase/RConn1 -- MOSFET LOWER/LConn1
  MOSFET UPPER/LConn1 -- D/RConn1

== system gmp_pmsm_sensored_nonlinear_sil_mdl_2022b/Three Phase Driver Model (Universal)/Single Phase Full Bridge V ==
  Enable : Inport
  PWM CMP : Inport  Port=2
  MOSFET LOWER : spsMosfetLib/Mosfet  Ron=R_mosfet_on  Lon=Lon  Rd=Rd  Vfd=Vf  IC=0  Rs=Rs  Cs=Cs  Measurements=off
  MOSFET UPPER : spsMosfetLib/Mosfet  Ron=R_mosfet_on  Lon=Lon  Rd=Rd  Vfd=Vf  IC=0  Rs=Rs  Cs=Cs  Measurements=off
  Triangle PWM modulation (with deadband)1 : Subsystem  mask{fswitch=fswitch, CMP_MAX=CMP_MAX, Deadband_Upper=Deadband_Upper, Deadband_Lower=Deadband_Lower, Deadband_us=NaN, phase_shift=phase_shift}
      mask prompts: Deadband_us "Deadband Time: (μs)"
      mask init:
      | calculate_deadband(gcb, 'Deadband_Upper', 'Deadband_Lower',	'CMP_MAX', 'fswitch', 'Deadband_us');
      mask Callback fswitch: calculate_deadband(gcb, 'Deadband_Upper', 'Deadband_Lower',	'CMP_MAX', 'fswitch', 'Deadband_us');
      mask Callback CMP_MAX: calculate_deadband(gcb, 'Deadband_Upper', 'Deadband_Lower',	'CMP_MAX', 'fswitch', 'Deadband_us');
      mask Callback Deadband_Upper:
      | calculate_deadband(gcb, 'Deadband_Upper', 'Deadband_Lower',	'CMP_MAX', 'fswitch', 'Deadband_us');
      | 
      | % Get handle of Mask
      | %mask_obj = Simulink.Mask.get(gcb);
      | %Parameters = Simulink.Mask.get(gcb).Parameters;
      | 
      | % Get source data
      | %dead_band_up = str2double(Parameters(strcmp(get_param(gcb,'MaskNames'),'Deadband_Upper')==1).Value);
      | %dead_band_dn = str2double(Parameters(strcmp(get_param(gcb,'MaskNames'),'Deadband_Lower')==1).Value);
      | %cmp_max = str2double(Parameters(strcmp(get_param(gcb,'MaskNames'),'CMP_MAX')==1).Value);
      | %switch_freq = str2double(Parameters(strcmp(get_param(gcb,'MaskNames'),'fswitch')==1).Value);
      | 
      | % calculate deadband
      | %dead_band_us = 1/switch_freq * (dead_band_up + dead_band_dn) / cmp_max*1e6;
      | 
      | % Set result
      | %Parameters(strcmp(get_param(gcb,'MaskNames'),'Deadband_upper_us')==1).Value=num2str(dead_band_us);
      mask Callback Deadband_Lower: calculate_deadband(gcb, 'Deadband_Upper', 'Deadband_Lower',	'CMP_MAX', 'fswitch', 'Deadband_upper_us');
      mask DialogControl DescGroupVar Prompt: PWM Modulator
      mask DialogControl Control8 Prompt: GMP CTL Simulink Utilities: virtual peripherals
      mask DialogControl DescTextVar Prompt: PWM Modulator. Input PWM compare register value, output ADC trigger signal, PWM output and negtive PWM output.
      mask DialogControl ParameterGroupVar Prompt: 参数
      mask DialogControl Control2 Prompt: PWM Frequency (Hz) :
      mask DialogControl Control4 Prompt: Full Scale PWM Compare value:
      mask DialogControl Control5 Prompt: (whole period is 2 * CMP_MAX ticks)
      mask DialogControl Control3 Prompt: Deadband Range Set (CMP Value):
      mask DialogControl Control6 Prompt: Single side deadband time: DEADBAND_CMP/2/CMP_MAX/fswitch
      mask DialogControl Control7 Prompt: Initial Phase (rad)
  D : PMIOPort  Side=Left
  Phase : PMIOPort  Port=2  Side=Right
  S : PMIOPort  Port=3  Side=Right
  Sample Trigger Output : Outport
  wires:
  PWM CMP/1 -> Triangle PWM modulation (with deadband)1/2(PWM CMP)
  Triangle PWM modulation (with deadband)1/2(PWM OUTPUT N) -> MOSFET LOWER/1
  Triangle PWM modulation (with deadband)1/3(Sample Trigger Output) -> Sample Trigger Output/1
  Enable/1 -> Triangle PWM modulation (with deadband)1/1(Enable)
  Triangle PWM modulation (with deadband)1/1(PWM OUTPUT) -> MOSFET UPPER/1
  connections:
  MOSFET LOWER/RConn1 -- S/RConn1
  MOSFET UPPER/RConn1 -- Phase/RConn1 -- MOSFET LOWER/LConn1
  MOSFET UPPER/LConn1 -- D/RConn1

== system gmp_pmsm_sensored_nonlinear_sil_mdl_2022b/Three Phase Driver Model (Universal)/Single Phase Full Bridge W ==
  Enable : Inport
  PWM CMP : Inport  Port=2
  MOSFET LOWER : spsMosfetLib/Mosfet  Ron=R_mosfet_on  Lon=Lon  Rd=Rd  Vfd=Vf  IC=0  Rs=Rs  Cs=Cs  Measurements=off
  MOSFET UPPER : spsMosfetLib/Mosfet  Ron=R_mosfet_on  Lon=Lon  Rd=Rd  Vfd=Vf  IC=0  Rs=Rs  Cs=Cs  Measurements=off
  Triangle PWM modulation (with deadband)1 : Subsystem  mask{fswitch=fswitch, CMP_MAX=CMP_MAX, Deadband_Upper=Deadband_Upper, Deadband_Lower=Deadband_Lower, Deadband_us=NaN, phase_shift=phase_shift}
      mask prompts: Deadband_us "Deadband Time: (μs)"
      mask init:
      | calculate_deadband(gcb, 'Deadband_Upper', 'Deadband_Lower',	'CMP_MAX', 'fswitch', 'Deadband_us');
      mask Callback fswitch: calculate_deadband(gcb, 'Deadband_Upper', 'Deadband_Lower',	'CMP_MAX', 'fswitch', 'Deadband_us');
      mask Callback CMP_MAX: calculate_deadband(gcb, 'Deadband_Upper', 'Deadband_Lower',	'CMP_MAX', 'fswitch', 'Deadband_us');
      mask Callback Deadband_Upper:
      | calculate_deadband(gcb, 'Deadband_Upper', 'Deadband_Lower',	'CMP_MAX', 'fswitch', 'Deadband_us');
      | 
      | % Get handle of Mask
      | %mask_obj = Simulink.Mask.get(gcb);
      | %Parameters = Simulink.Mask.get(gcb).Parameters;
      | 
      | % Get source data
      | %dead_band_up = str2double(Parameters(strcmp(get_param(gcb,'MaskNames'),'Deadband_Upper')==1).Value);
      | %dead_band_dn = str2double(Parameters(strcmp(get_param(gcb,'MaskNames'),'Deadband_Lower')==1).Value);
      | %cmp_max = str2double(Parameters(strcmp(get_param(gcb,'MaskNames'),'CMP_MAX')==1).Value);
      | %switch_freq = str2double(Parameters(strcmp(get_param(gcb,'MaskNames'),'fswitch')==1).Value);
      | 
      | % calculate deadband
      | %dead_band_us = 1/switch_freq * (dead_band_up + dead_band_dn) / cmp_max*1e6;
      | 
      | % Set result
      | %Parameters(strcmp(get_param(gcb,'MaskNames'),'Deadband_upper_us')==1).Value=num2str(dead_band_us);
      mask Callback Deadband_Lower: calculate_deadband(gcb, 'Deadband_Upper', 'Deadband_Lower',	'CMP_MAX', 'fswitch', 'Deadband_upper_us');
      mask DialogControl DescGroupVar Prompt: PWM Modulator
      mask DialogControl Control8 Prompt: GMP CTL Simulink Utilities: virtual peripherals
      mask DialogControl DescTextVar Prompt: PWM Modulator. Input PWM compare register value, output ADC trigger signal, PWM output and negtive PWM output.
      mask DialogControl ParameterGroupVar Prompt: 参数
      mask DialogControl Control2 Prompt: PWM Frequency (Hz) :
      mask DialogControl Control4 Prompt: Full Scale PWM Compare value:
      mask DialogControl Control5 Prompt: (whole period is 2 * CMP_MAX ticks)
      mask DialogControl Control3 Prompt: Deadband Range Set (CMP Value):
      mask DialogControl Control6 Prompt: Single side deadband time: DEADBAND_CMP/2/CMP_MAX/fswitch
      mask DialogControl Control7 Prompt: Initial Phase (rad)
  D : PMIOPort  Side=Left
  Phase : PMIOPort  Port=2  Side=Right
  S : PMIOPort  Port=3  Side=Right
  Sample Trigger Output : Outport
  wires:
  PWM CMP/1 -> Triangle PWM modulation (with deadband)1/2(PWM CMP)
  Triangle PWM modulation (with deadband)1/2(PWM OUTPUT N) -> MOSFET LOWER/1
  Triangle PWM modulation (with deadband)1/3(Sample Trigger Output) -> Sample Trigger Output/1
  Enable/1 -> Triangle PWM modulation (with deadband)1/1(Enable)
  Triangle PWM modulation (with deadband)1/1(PWM OUTPUT) -> MOSFET UPPER/1
  connections:
  MOSFET LOWER/RConn1 -- S/RConn1
  MOSFET UPPER/RConn1 -- Phase/RConn1 -- MOSFET LOWER/LConn1
  MOSFET UPPER/LConn1 -- D/RConn1

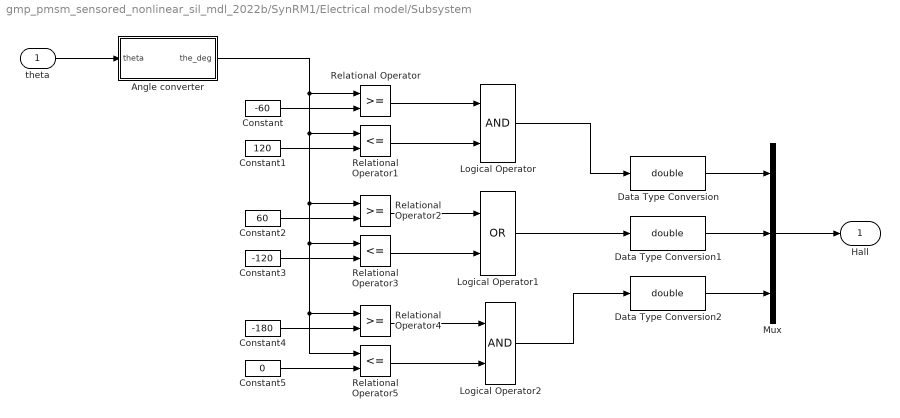
== system gmp_pmsm_sensored_nonlinear_sil_mdl_2022b/SynRM1/Electrical model/Subsystem ==
  theta : Inport
  Angle converter : Subsystem
  Constant : Constant  Value=-60
  Constant1 : Constant  Value=120
  Constant2 : Constant  Value=60
  Constant3 : Constant  Value=-120
  Constant4 : Constant  Value=-180
  Constant5 : Constant  Value=0
  Data Type Conversion : DataTypeConversion  OutDataTypeStr=double  SaturateOnIntegerOverflow=off
  Data Type Conversion1 : DataTypeConversion  OutDataTypeStr=double  SaturateOnIntegerOverflow=off
  Data Type Conversion2 : DataTypeConversion  OutDataTypeStr=double  SaturateOnIntegerOverflow=off
  Logical Operator : Logic  AllPortsSameDT=off  OutDataTypeStr=boolean
  Logical Operator1 : Logic  Operator=OR  AllPortsSameDT=off  OutDataTypeStr=boolean
  Logical Operator2 : Logic  AllPortsSameDT=off  OutDataTypeStr=boolean
  Mux : Mux  Inputs=3
  Relational Operator : RelationalOperator  OutDataTypeStr=boolean  RndMeth=Simplest  InputSameDT=off
  Relational Operator1 : RelationalOperator  Operator=<=  OutDataTypeStr=boolean  RndMeth=Simplest  InputSameDT=off
  Relational Operator2 : RelationalOperator  OutDataTypeStr=boolean  RndMeth=Simplest  InputSameDT=off
  Relational Operator3 : RelationalOperator  Operator=<=  OutDataTypeStr=boolean  RndMeth=Simplest  InputSameDT=off
  Relational Operator4 : RelationalOperator  OutDataTypeStr=boolean  RndMeth=Simplest  InputSameDT=off
  Relational Operator5 : RelationalOperator  Operator=<=  OutDataTypeStr=boolean  RndMeth=Simplest  InputSameDT=off
  Hall : Outport  VectorParamsAs1DForOutWhenUnconnected=off
  wires:
  theta/1 -> Angle converter/1(theta)
  Mux/1 -> Hall/1
  Data Type Conversion1/1 -> Mux/2
  Data Type Conversion/1 -> Mux/1
  Data Type Conversion2/1 -> Mux/3
  Logical Operator/1 -> Data Type Conversion/1
  Logical Operator2/1 -> Data Type Conversion2/1
  Logical Operator1/1 -> Data Type Conversion1/1
  Constant1/1 -> Relational Operator1/2
  Constant/1 -> Relational Operator/2
  Constant4/1 -> Relational Operator4/2
  Constant5/1 -> Relational Operator5/2
  Angle converter/1(the_deg) -> Relational Operator1/1, Relational Operator5/1, Relational Operator4/1, Relational Operator3/1, Relational Operator2/1, Relational Operator/1
  Constant2/1 -> Relational Operator2/2
  Constant3/1 -> Relational Operator3/2
  Relational Operator3/1 -> Logical Operator1/2
  Relational Operator2/1 -> Logical Operator1/1
  Relational Operator/1 -> Logical Operator/1
  Relational Operator1/1 -> Logical Operator/2
  Relational Operator4/1 -> Logical Operator2/1
  Relational Operator5/1 -> Logical Operator2/2

== system gmp_pmsm_sensored_nonlinear_sil_mdl_2022b/SynRM1/Electrical model/Subsystem1 ==
  theta : Inport
  s,c : Inport  Port=2
  iq,id : Inport  Port=3
  Add : Sum  Commented=on  Inputs=--
  Constant : Constant  Value=0
  Demux : Demux  Outputs=2
  Fcn : Fcn  Commented=on  Expr=u[3]*u[2] + u[4]*u[1]
  Fcn1 : Fcn  Commented=on  Expr=(u[2]*(-u[3]-sqrt(3)*u[4]) + u[1] * (sqrt(3)*u[3]-u[4])) * 0.5
  Mux : Mux  Commented=on  Inputs=[2, 2]
  Mux1 : Mux  Commented=on  Inputs=3
  Mux2 : Mux  Inputs=3
  dq0 to abc : spsdq0toabcLib/dq0 to abc  Alignment=Aligned with phase A axis
  is : Outport  VectorParamsAs1DForOutWhenUnconnected=off
  wires:
  s,c/1 -> Mux/1
  iq,id/1 -> Demux/1
  Fcn/1 -> Add/2, Mux1/1
  Fcn1/1 -> Add/1, Mux1/2
  Add/1 -> Mux1/3
  Mux/1 -> Fcn1/1, Fcn/1
  Mux1/1 -> ?
  theta/1 -> dq0 to abc/2
  Demux/1 -> Mux2/2
  Demux/2 -> Mux2/1
  Mux2/1 -> dq0 to abc/1
  dq0 to abc/1 -> is/1
  Constant/1 -> Mux2/3

== system gmp_pmsm_sensored_nonlinear_sil_mdl_2022b/SynRM1/Electrical model/Subsystem2 ==
  vq,vd : Inport
  we : Inport  Port=2
  LdLqRWb : Inport  Port=3
  Demux : Demux  Outputs=2
  Mux : Mux  Inputs=2
  Mux1 : Mux  Inputs=2
  id : Subsystem
  iq : Subsystem
  iq,id : Outport  VectorParamsAs1DForOutWhenUnconnected=off
  p_idiq_con : Outport  Port=2
  wires:
  Demux/1 -> iq/1(vq)
  id/1(id) -> iq/3(id), Mux/2
  we/1 -> iq/2(we), id/2(we)
  iq/1(iq) -> id/1(iq), Mux/1
  LdLqRWb/1 -> iq/4(LdLqRWb), id/4(LdLqRWb)
  Demux/2 -> id/3(vd)
  Mux/1 -> iq,id/1
  vq,vd/1 -> Demux/1
  iq/2(p_iq_con) -> Mux1/2
  id/2(p_id_con) -> Mux1/1
  Mux1/1 -> p_idiq_con/1

== system gmp_pmsm_sensored_nonlinear_sil_mdl_2022b/SynRM1/Electrical model/abc2qd ==
  "Vab, Vbc" : Inport
  theta : Inport  Port=2
  Mux : Mux  Inputs=2
  Mux1 : Mux  Inputs=[2, 2]
  Mux2 : Mux  Inputs=2
  Trigonometric Function : Trigonometry
  Trigonometric Function1 : Trigonometry  Operator=cos
  Vd : Fcn  Expr=( u[4]*(2*u[1]+u[2]) + (sqrt(3)*u[2]*u[3]) ) * 1/3
  Vq : Fcn  Expr=( -u[3]*(2*u[1]+u[2]) + (sqrt(3)*u[2]*u[4]) ) * 1/3
  "s, c" : Outport  VectorParamsAs1DForOutWhenUnconnected=off
  "vq, vd" : Outport  Port=2  VectorParamsAs1DForOutWhenUnconnected=off
  wires:
  Mux1/1 -> Vd/1, Vq/1
  Vd/1 -> Mux2/2
  Vq/1 -> Mux2/1
  Trigonometric Function/1 -> Mux/1
  Mux2/1 -> "vq, vd"/1
  Mux/1 -> "s, c"/1, Mux1/2
  theta/1 -> Trigonometric Function1/1, Trigonometric Function/1
  Trigonometric Function1/1 -> Mux/2
  "Vab, Vbc"/1 -> Mux1/1

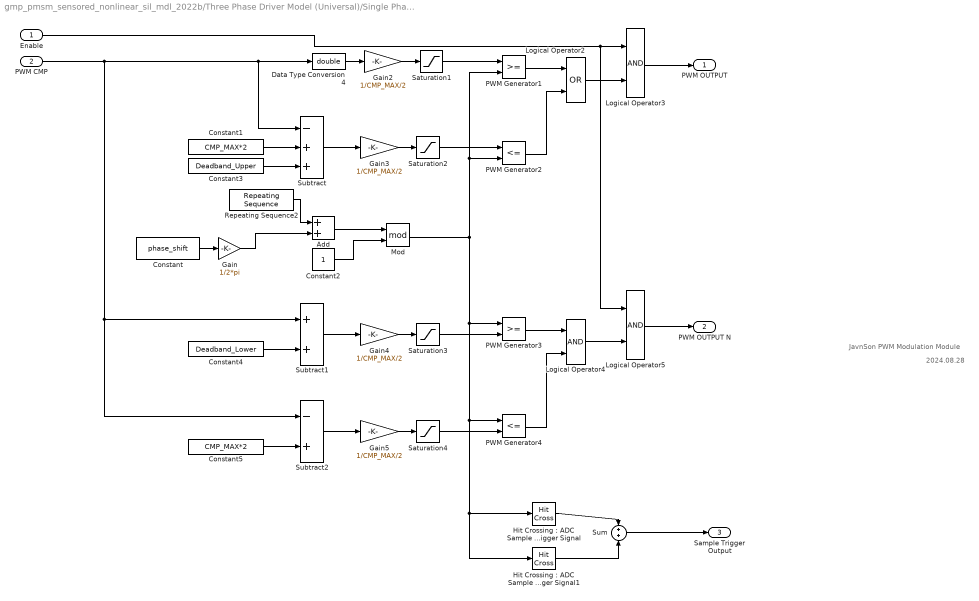
== system gmp_pmsm_sensored_nonlinear_sil_mdl_2022b/Three Phase Driver Model (Universal)/Single Phase Full Bridge U/Triangle PWM modulation (with deadband)1 ==
  note: JavnSon PWM Modulation Module
  note: 2024.08.28
  Enable : Inport
  PWM CMP : Inport  Port=2
  Add : Sum
  Constant : Constant  Value=phase_shift
  Constant1 : Constant  Value=CMP_MAX*2
  Constant2 : Constant
  Constant3 : Constant  Value=Deadband_Upper
  Constant4 : Constant  Value=Deadband_Lower
  Constant5 : Constant  Value=CMP_MAX*2
  Data Type Conversion4 : DataTypeConversion  OutDataTypeStr=double  SaturateOnIntegerOverflow=off  RndMeth=Floor
  Gain : Gain  Gain=1/2*pi
  Gain{2..5} (4 alike) : Gain  Gain=1/CMP_MAX/2
  Hit Crossing：ADC Sample Trigger Signal : HitCross  HitCrossingOffset=0.5  HitCrossingDirection=rising
  Hit Crossing：ADC Sample Trigger Signal1 : HitCross  HitCrossingOffset=0.5  HitCrossingDirection=falling
  Logical Operator2 : Logic  Operator=OR  AllPortsSameDT=off  OutDataTypeStr=boolean
  Logical Operator3 : Logic  AllPortsSameDT=off  OutDataTypeStr=boolean
  Logical Operator4 : Logic  AllPortsSameDT=off  OutDataTypeStr=boolean
  Logical Operator5 : Logic  AllPortsSameDT=off  OutDataTypeStr=boolean
  Mod : Math  Operator=mod
  PWM Generator1 : RelationalOperator  OutDataTypeStr=boolean  InputSameDT=off
  PWM Generator2 : RelationalOperator  Operator=<=  OutDataTypeStr=boolean  InputSameDT=off
  PWM Generator3 : RelationalOperator  OutDataTypeStr=boolean  InputSameDT=off
  PWM Generator4 : RelationalOperator  Operator=<=  OutDataTypeStr=boolean  InputSameDT=off
  Repeating Sequence2 : simulink/Sources/Repeating Sequence  rep_seq_t=[0, 1/2/fswitch, 1/fswitch ]  rep_seq_y=[0,0.5,1]
  Saturation{1..4} (4 alike) : Saturate  UpperLimit=1  LowerLimit=0
  Subtract : Sum  Inputs=-++
  Subtract1 : Sum
  Subtract2 : Sum  Inputs=-+
  Sum : Sum  Inputs=+|+
  PWM OUTPUT : Outport
  PWM OUTPUT N : Outport  Port=2
  Sample Trigger Output : Outport  Port=3
  wires:
  Constant/1 -> Gain/1
  Constant2/1 -> Mod/2
  Add/1 -> Mod/1
  Gain/1 -> Add/2
  Repeating Sequence2/1 -> Add/1
  Logical Operator3/1 -> PWM OUTPUT/1
  Logical Operator5/1 -> PWM OUTPUT N/1
  Enable/1 -> Logical Operator3/1, Logical Operator5/1
  Mod/1 -> PWM Generator4/1, Hit Crossing：ADC Sample Trigger Signal1/1, Hit Crossing：ADC Sample Trigger Signal/1, PWM Generator3/1, PWM Generator1/2, PWM Generator2/2
  Logical Operator4/1 -> Logical Operator5/2
  PWM Generator4/1 -> Logical Operator4/2
  Subtract2/1 -> Gain5/1
  Gain5/1 -> Saturation4/1
  Saturation4/1 -> PWM Generator4/2
  Constant5/1 -> Subtract2/2
  PWM Generator3/1 -> Logical Operator4/1
  Saturation3/1 -> PWM Generator3/2
  Subtract1/1 -> Gain4/1
  Gain4/1 -> Saturation3/1
  Constant4/1 -> Subtract1/2
  Saturation2/1 -> PWM Generator2/1
  Subtract/1 -> Gain3/1
  Gain3/1 -> Saturation2/1
  PWM Generator2/1 -> Logical Operator2/2
  Constant3/1 -> Subtract/3
  Constant1/1 -> Subtract/2
  Logical Operator2/1 -> Logical Operator3/2
  PWM Generator1/1 -> Logical Operator2/1
  Saturation1/1 -> PWM Generator1/1
  Gain2/1 -> Saturation1/1
  Data Type Conversion4/1 -> Gain2/1
  PWM CMP/1 -> Data Type Conversion4/1, Subtract/1, Subtract1/1, Subtract2/1
  Sum/1 -> Sample Trigger Output/1
  Hit Crossing：ADC Sample Trigger Signal/1 -> Sum/1
  Hit Crossing：ADC Sample Trigger Signal1/1 -> Sum/2
